simulink model "Transfer_Function"  (R2024b)
settings: Solver=FixedStepAuto  StartTime=0.0  StopTime=inf  FixedStep=0.01  RelTol=1e-3  EnableMultiTasking=on
libraries: arduinolib x12
settings Model: ExtModeTrigDuration=2  Creator=devan  LastModifiedBy=devan
settings SolverCC: AutoInsertRateTranBlk=on
settings OptimizationCC: EnhancedBackFolding=on  PassReuseOutputArgsAs=Individual arguments  ZeroExternalMemoryAtStartup=off  ZeroInternalMemoryAtStartup=off  MaxStackSize=64  OptimizeBlockOrder=speed  DifferentSizesBufferReuse=on  OptimizationCustomize=off  EfficientTunableParamExpr=on
settings DebuggingCC: ParameterTunabilityLossMsg=error
settings HardwareCC: ProdBitPerInt=16  ProdBitPerPointer=16  ProdBitPerSizeT=16  ProdBitPerPtrDiffT=16  ProdLargestAtomicFloat=None  ProdWordSize=8  ProdHWDeviceType=Atmel->AVR  UseEmbeddedCoderFeatures=off
settings SFSimCC: MATLABDynamicMemAlloc=off
settings RTWCC: Description=Embedded Coder  SystemTargetFile=ert.tlc  HardwareBoard=Arduino Nano 3.0  TemplateMakefile=ert_default_tmf  Toolchain=Arduino AVR  BuildConfiguration=Faster Runs
settings CodeAppCC: ForceParamTrailComments=on  IgnoreCustomStorageClasses=off  OperatorAnnotations=on  SimulinkDataObjDesc=on  SFDataObjDesc=on  InsertBlockDesc=on
settings ERTTargetCC: SupportContinuousTime=on  SupportNonInlinedSFcns=on  SupportVariableSizeSignals=on  ExtModeTransport=3  ExtModeStaticAlloc=on  ExtModeAutomaticAllocSize=off  ExtModeStaticAllocSize=250  ExtModeMexFile=ext_xcp  ExtModeIntrfLevel=Level2 - Open  InlinedParameterPlacement=Hierarchical

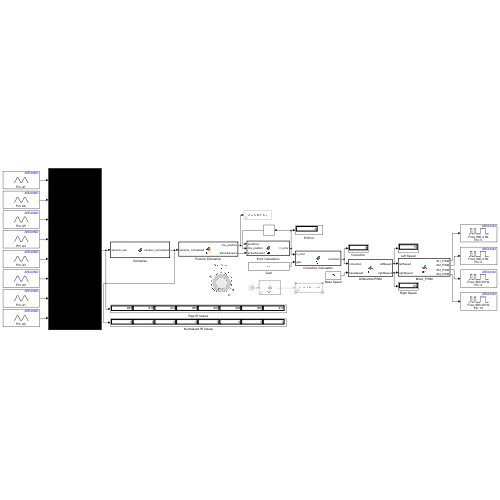
[thumbnail: Simulink's stored preview of the top-level diagram]
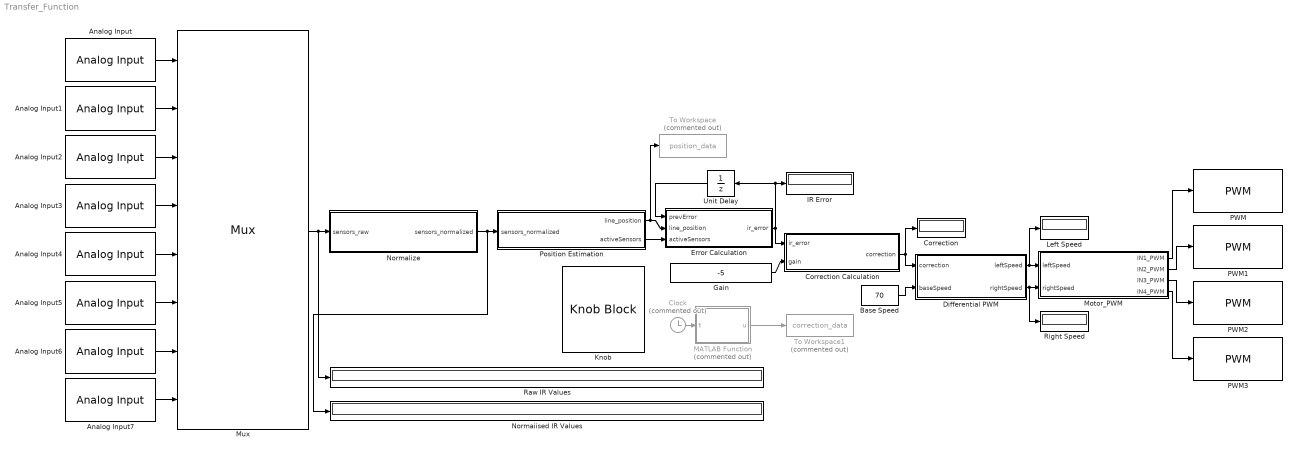
== system Transfer_Function ==
  Analog Input : arduinolib/Analog Input  pinNumber=7  ReadResultsOnly=off  ConversionTriggerSource=Software  ExternalTriggerType=uint32( 0 )  OutputDataType=uint16  EnableConversionCompleteNotify=off  EnableOuputStatus=off  SampleTime=0.01  blockPlatform=arduino
      settings: SourceProductName=Common
  Analog Input1 : arduinolib/Analog Input  pinNumber=6  ReadResultsOnly=off  ConversionTriggerSource=Software  ExternalTriggerType=uint32( 0 )  OutputDataType=uint16  EnableConversionCompleteNotify=off  EnableOuputStatus=off  SampleTime=0.01  blockPlatform=arduino
      settings: SourceProductName=Common
  Analog Input2 : arduinolib/Analog Input  pinNumber=5  ReadResultsOnly=off  ConversionTriggerSource=Software  ExternalTriggerType=uint32( 0 )  OutputDataType=uint16  EnableConversionCompleteNotify=off  EnableOuputStatus=off  SampleTime=0.01  blockPlatform=arduino
      settings: SourceProductName=Common
  Analog Input3 : arduinolib/Analog Input  pinNumber=4  ReadResultsOnly=off  ConversionTriggerSource=Software  ExternalTriggerType=uint32( 0 )  OutputDataType=uint16  EnableConversionCompleteNotify=off  EnableOuputStatus=off  SampleTime=0.01  blockPlatform=arduino
      settings: SourceProductName=Common
  Analog Input4 : arduinolib/Analog Input  pinNumber=3  ReadResultsOnly=off  ConversionTriggerSource=Software  ExternalTriggerType=uint32( 0 )  OutputDataType=uint16  EnableConversionCompleteNotify=off  EnableOuputStatus=off  SampleTime=0.01  blockPlatform=arduino
      settings: SourceProductName=Common
  Analog Input5 : arduinolib/Analog Input  pinNumber=2  ReadResultsOnly=off  ConversionTriggerSource=Software  ExternalTriggerType=uint32( 0 )  OutputDataType=uint16  EnableConversionCompleteNotify=off  EnableOuputStatus=off  SampleTime=0.01  blockPlatform=arduino
      settings: SourceProductName=Common
  Analog Input6 : arduinolib/Analog Input  pinNumber=1  ReadResultsOnly=off  ConversionTriggerSource=Software  ExternalTriggerType=uint32( 0 )  OutputDataType=uint16  EnableConversionCompleteNotify=off  EnableOuputStatus=off  SampleTime=0.01  blockPlatform=arduino
      settings: SourceProductName=Common
  Analog Input7 : arduinolib/Analog Input  pinNumber=0  ReadResultsOnly=off  ConversionTriggerSource=Software  ExternalTriggerType=uint32( 0 )  OutputDataType=uint16  EnableConversionCompleteNotify=off  EnableOuputStatus=off  SampleTime=0.01  blockPlatform=arduino
      settings: SourceProductName=Common
  Base Speed : Constant  Value=70
  Clock : Clock  Commented=on
  Correction : Display
  Correction Calculation : MATLAB Function  TreatAsAtomicUnit=on
  Differential PWM : MATLAB Function  TreatAsAtomicUnit=on
  Error Calculation : MATLAB Function  TreatAsAtomicUnit=on
  Gain : Constant  Value=-5
  IR Error : Display
  Knob : KnobBlock  ScaleMax=10
  Left Speed : Display
  MATLAB Function : MATLAB Function  Commented=on  TreatAsAtomicUnit=on
  Motor_PWM : MATLAB Function  TreatAsAtomicUnit=on
  Mux : Mux  Inputs=8
  Normaiised IR Values : Display
  Normalize : MATLAB Function  TreatAsAtomicUnit=on
  PWM : arduinolib/PWM  pinNumber=5  frequencyType=Specify  desiredFrequency=980.4  achievableFrequency=980.4
      settings: SourceProductName=Common
  PWM1 : arduinolib/PWM  pinNumber=6  frequencyType=Specify  desiredFrequency=980.4  achievableFrequency=980.4
      settings: SourceProductName=Common
  PWM2 : arduinolib/PWM  pinNumber=9  frequencyType=Specify  desiredFrequency=980.4  achievableFrequency=980.3922
      settings: SourceProductName=Common
  PWM3 : arduinolib/PWM  pinNumber=10  frequencyType=Specify  desiredFrequency=980.4  achievableFrequency=980.3922
      settings: SourceProductName=Common
  Position Estimation : MATLAB Function  TreatAsAtomicUnit=on
  Raw IR Values : Display
  Right Speed : Display
  To Workspace : ToWorkspace  Commented=on  VariableName=position_data  SaveFormat=Timeseries  SampleTime=-1
  To Workspace1 : ToWorkspace  Commented=on  VariableName=correction_data  SaveFormat=Timeseries  SampleTime=-1
  Unit Delay : UnitDelay  SampleTime=-1  HasFrameUpgradeWarning=on
  wires:
  Analog Input/1 -> Mux/1
  Analog Input1/1 -> Mux/2
  Analog Input2/1 -> Mux/3
  Analog Input3/1 -> Mux/4
  Analog Input4/1 -> Mux/5
  Analog Input5/1 -> Mux/6
  Analog Input6/1 -> Mux/7
  Analog Input7/1 -> Mux/8
  Mux/1 -> Raw IR Values/1, Normalize/1(sensors_raw)
  Normalize/1(sensors_normalized) -> Normaiised IR Values/1, Position Estimation/1(sensors_normalized)
  Position Estimation/1(line_position) -> To Workspace/1, Error Calculation/2(line_position)
  Position Estimation/2(activeSensors) -> Error Calculation/3(activeSensors)
  Error Calculation/1(ir_error) -> IR Error/1, Unit Delay/1, Correction Calculation/1(ir_error)
  Correction Calculation/1(correction) -> Correction/1, Differential PWM/1(correction)
  Base Speed/1 -> Differential PWM/2(baseSpeed)
  Differential PWM/1(leftSpeed) -> Left Speed/1, Motor_PWM/1(leftSpeed)
  Differential PWM/2(rightSpeed) -> Right Speed/1, Motor_PWM/2(rightSpeed)
  Motor_PWM/1(IN1_PWM) -> PWM/1
  Motor_PWM/2(IN2_PWM) -> PWM1/1
  Motor_PWM/3(IN3_PWM) -> PWM2/1
  Motor_PWM/4(IN4_PWM) -> PWM3/1
  Unit Delay/1 -> Error Calculation/1(prevError)
  Clock/1 -> MATLAB Function/1(t)
  MATLAB Function/1(u) -> To Workspace1/1
  Gain/1 -> Correction Calculation/2(gain)

== matlab function Transfer_Function/Normalize ==
  data: sensors_raw input; sensors_normalized output
function sensors_normalized = fcn(sensors_raw)

    sensors_normalized = sensors_raw < 500;

end

== matlab function Transfer_Function/Position Estimation ==
  data: sensors_normalized input; line_position output; activeSensors output
function [line_position, activeSensors] = fcn(sensors_normalized)

    weights = [-3, -2, -1, 0, 0, 1, 2, 3];
    line_position = 0;
    activeSensors = 0;

    for i = 1 : length(sensors_normalized)

        if sensors_normalized(i) == 1
            activeSensors = activeSensors + 1;
        end

        line_position = line_position + sensors_normalized(i) * weights(i);
    end

end

== matlab function Transfer_Function/Error Calculation ==
  data: prevError input; line_position input; ir_error output; activeSensors input
function ir_error = fcn(prevError, line_position, activeSensors)

    if activeSensors == 0
        if prevError > 0
            line_position = 12;
        else
            line_position = -12;
        end
    end
    
    ir_error = line_position / 2;
end

== matlab function Transfer_Function/Correction Calculation ==
  data: correction output; ir_error input; gain input
function correction = fcn(ir_error, gain)

    % correction = gain * ir_error;
    correction = gain;

end

== matlab function Transfer_Function/Differential PWM ==
  data: correction input; leftSpeed output; baseSpeed input; rightSpeed output
function [leftSpeed,rightSpeed] = fcn(correction, baseSpeed)

leftSpeed = min(max(baseSpeed - correction,-255),255);
rightSpeed = min(max(baseSpeed + correction,-255),255);

end

== matlab function Transfer_Function/Motor_PWM ==
  data: leftSpeed input; IN1_PWM output; rightSpeed input; IN2_PWM output; IN3_PWM output; IN4_PWM output
function [IN1_PWM, IN2_PWM, IN3_PWM, IN4_PWM] = fcn(leftSpeed, rightSpeed)

leftSpeed  = min(max(leftSpeed, -255), 255);
rightSpeed = min(max(rightSpeed, -255), 255);

IN1_PWM = 0;
IN2_PWM = 0;
IN3_PWM = 0;
IN4_PWM = 0;

if leftSpeed >= 0
    IN1_PWM = leftSpeed;
    IN2_PWM = 0;
else
    IN1_PWM = 0;
    IN2_PWM = -leftSpeed;
end

if rightSpeed >= 0
    IN3_PWM = rightSpeed;
    IN4_PWM = 0;
else
    IN3_PWM = 0;
    IN4_PWM = -rightSpeed;
end

== matlab function Transfer_Function/MATLAB Function ==
  data: t input; u output
function u = fcn(t)

var = 1;

if t == 0
    u = 0;
elseif t < 0.25
    u = var;
elseif t < 0.5
    u = 0;
elseif t < 0.75
    u = -var;
elseif t < 1
    u = 0;
elseif t < 1.25
    u = -2 * var;
elseif t < 1.5
    u = 0;
elseif t < 1.75
    u = 2 * var;
else
    u = 0;
end
